simulink model "Drive_DC"  (R2022b)
settings: Solver=VariableStepAuto  StartTime=0.0  StopTime=13  MaxStep=1e-5  RelTol=1e-3
undefined symbols (not defined in the file or in its folder): DiscIntNeverNeededParam, sigbuilder_block
libraries: spsMeanLib x6, slpidlib x5, simulink_extras x5, spsSawtoothGeneratorLib x4, simulink x2, pid_lib x1, spspowerguiLib x1
(part 2 of 2)

== system Drive_DC/Dual_Rectifier_Control/Speed_Control ==
  note: PI_system3
  In1 : Inport
  In2 : Inport  Port=2
  AND : Logic  Operator=NAND  AllPortsSameDT=off  OutDataTypeStr=boolean
  Discrete-Time Integrator : DiscreteIntegrator  SampleTime=-1  ICPrevOutput=DiscIntNeverNeededParam  ICPrevScaledInput=DiscIntNeverNeededParam
  Equal : RelationalOperator  Operator=~=  OutDataTypeStr=boolean  RndMeth=Simplest  InputSameDT=off
  Equal1 : RelationalOperator  Operator===  OutDataTypeStr=boolean  RndMeth=Simplest  InputSameDT=off
  KI : Gain  Gain=0.5
  Kp : Gain  Gain=0.5
  PID Controller : slpidlib/PID Controller  Commented=on  Controller=PI  Form=Parallel  TimeDomain=Continuous-time  UseExternalTs=off  SampleTime=-1  IntegratorMethod=Forward Euler  FilterMethod=Forward Euler  ControllerParametersSource=internal  P=0.5  I=0.5  UseKiTs=off  D=0  N=100  UseFilter=on  TunerSelectOption=Transfer Function Based (PID Tuner App)  InitialConditionSource=internal  InitialConditionForIntegrator=0  InitialConditionForFilter=0  DifferentiatorICPrevScaledInput=0  ExternalReset=none  TrackingMode=off  Kt=1  LimitOutput=on  SatLimitsSource=internal  UpperSaturationLimit=(30*746)/(1740*pi/30)  LowerSaturationLimit=-(30*746)/(1740*pi/30)  LinearizeAsGain=on  AntiWindupMode=clamping  Kb=1  LimitIntegrator=off  UpperIntegratorSaturationLimit=inf  LowerIntegratorSaturationLimit=-inf  POutMin=[]  POutMax=[]  IOutMin=[]  IOutMax=[]  DOutMin=[]  DOutMax=[]  NOutMin=[]  NOutMax=[]  SumOutMin=[]  SumOutMax=[]  SaturationOutMin=[]  SaturationOutMax=[]  PParamMin=[]  PParamMax=[]  IParamMin=[]  IParamMax=[]  DParamMin=[]  DParamMax=[]  NParamMin=[]  NParamMax=[]  KbParamMin=[]  KbParamMax=[]  KtParamMin=[]  KtParamMax=[]  KbOutMin=[]  KbOutMax=[]  KtOutMin=[]  KtOutMax=[]  IntegratorOutMin=[]  IntegratorOutMax=[]  FilterOutMin=[]  FilterOutMax=[]  SumI1OutMin=[]  SumI1OutMax=[]  SumI2OutMin=[]  SumI2OutMax=[]  SumI3OutMin=[]  SumI3OutMax=[]  SumI4OutMin=[]  SumI4OutMax=[]  SumDOutMin=[]  SumDOutMax=[]  DifferentiatorOutMin=[]  DifferentiatorOutMax=[]  FilterDiffOutCoefMin=[]  FilterDiffOutCoefMax=[]  ReciprocalOutMin=[]  ReciprocalOutMax=[]  SumDenOutMin=[]  SumDenOutMax=[]  SumNumOutMin=[]  SumNumOutMax=[]  DivideOutMin=[]  DivideOutMax=[]  UdiffTsProdOutMin=[]  UdiffTsProdOutMax=[]  NTsProdOutMin=[]  NTsProdOutMax=[]  UintegralTsProdOutMin=[]  UintegralTsProdOutMax=[]  UngainTsProdOutMin=[]  UngainTsProdOutMax=[]  ClampingZeroOutDataTypeStr=Inherit: Inherit via back propagation  ClampingZeroOutMin=[]  ClampingZeroOutMax=[]  FilterDenConstantOutDataTypeStr=Inherit: Inherit via back propagation  FilterDenConstantOutMin=[]  FilterDenConstantOutMax=[]  PCopyOutDataTypeStr=Inherit: Inherit via back propagation  PCopyOutMin=[]  PCopyOutMax=[]  NCopyOutDataTypeStr=Inherit: Inherit via back propagation  NCopyOutMin=[]  NCopyOutMax=[]  IntegratorContinuousStateAttributes=''  IntegratorStateMustResolveToSignalObject=off  IntegratorRTWStateStorageClass=Auto  FilterContinuousStateAttributes=''  FilterStateMustResolveToSignalObject=off  FilterRTWStateStorageClass=Auto  ParallelPVariant=InternalParameters  IdealPVariant=Disabled  IVariant=InternalParameters  DVariant=Disabled  IntegratorVariant=Continuous  SatVariant=Enabled  AWVariant=ContClampingParallel  PCopyVariant=Disabled  TRVariant=Disabled  FdbkBlocksVariant=Forward  IdealPFdbkVariant=Disabled  SatFdbkVariant=Disabled  DerivativeFilterVariant=Disabled  NVariant=Disabled  NCopyVariant=Disabled_SignalSpec  FilterICVariant=Disabled  IntegratorICVariant=InternalICs  ExternalResetVariant=Disabled  TRSumVariant=Passthrough  SumFdbkVariant=Disabled  SumVariant=Sum_PI  TsampFilterVariant=InternalTs  TsampNgainVariant=Passthrough  TsampIntegralVariant=Passthrough  ExternalSaturationOutDataTypeStr=Inherit: Same as second input
  Product : Product
  Saturation1 : Saturate  UpperLimit=(30*746)/(1740*pi/30)  LowerLimit=-(30*746)/(1740*pi/30)
  Sign : Signum
  Sign1 : Signum
  Sum : Sum  Inputs=|+-
  Sum2 : Sum  Inputs=|++
  Unit Delay : UnitDelay  SampleTime=-1  HasFrameUpgradeWarning=on
  Unit Delay1 : UnitDelay  SampleTime=-1  HasFrameUpgradeWarning=on
  Tref : Outport
  wires:
  In2/1 -> Sum/2
  In1/1 -> Sum/1
  Discrete-Time Integrator/1 -> Sum2/1
  Kp/1 -> Sum2/2
  KI/1 -> Discrete-Time Integrator/1
  Sum2/1 -> Saturation1/1, Unit Delay/1
  Saturation1/1 -> Tref/1, Unit Delay1/1
  Sign/1 -> Equal1/2
  Sign1/1 -> Equal1/1
  Equal1/1 -> AND/1
  Equal/1 -> AND/2
  Unit Delay/1 -> Equal/1, Sign/1
  Product/1 -> KI/1
  Unit Delay1/1 -> Equal/2
  AND/1 -> Product/1
  Sum/1 -> Kp/1, Sign1/1, Product/2

== system Drive_DC/Dual_Rectifier_Control/Subsystem5 ==
  Va : Inport
  Vf : Inport  Port=2
  Tl : Inport  Port=3
  Gain : Gain  Gain=Ra
  Gain1 : Gain  Gain=k
  Gain2 : Gain  Gain=1/La
  Gain3 : Gain  Gain=Rf
  Gain4 : Gain  Gain=1/Lf
  Gain5 : Gain  Gain=k
  Gain6 : Gain  Gain=1/J
  Integrator : Integrator
  Integrator1 : Integrator
  Integrator2 : Integrator
  Subtract : Sum  Inputs=+--
  Subtract1 : Sum  Inputs=+-
  Subtract2 : Sum  Inputs=+-
  Ia : Outport
  If : Outport  Port=2
  Te : Outport  Port=3
  Wm : Outport  Port=4
  wires:
  Gain6/1 -> Integrator2/1
  Subtract2/1 -> Gain6/1
  Tl/1 -> Subtract2/2
  Gain5/1 -> Te/1, Subtract2/1
  Gain3/1 -> Subtract1/2
  Integrator1/1 -> If/1, Gain3/1
  Subtract1/1 -> Gain4/1
  Gain4/1 -> Integrator1/1
  Vf/1 -> Subtract1/1
  Gain2/1 -> Integrator/1
  Subtract/1 -> Gain2/1
  Gain1/1 -> Subtract/3
  Integrator2/1 -> Wm/1, Gain1/1
  Gain/1 -> Subtract/2
  Va/1 -> Subtract/1
  Integrator/1 -> Gain/1, Ia/1, Gain5/1

== system Drive_DC/Subsystem4/Subsystem ==
  Va : Inport
  W : Inport  Port=2
  Gain : Gain  Gain=Ra
  Gain1 : Gain  Gain=k
  Gain2 : Gain  Gain=1/La
  Integrator : Integrator
  Subtract : Sum  Inputs=+--
  Ia : Outport
  wires:
  Subtract/1 -> Gain2/1
  Integrator/1 -> Ia/1, Gain/1
  Va/1 -> Subtract/1
  Gain/1 -> Subtract/2
  Gain2/1 -> Integrator/1
  Gain1/1 -> Subtract/3
  W/1 -> Gain1/1

== system Drive_DC/Subsystem4/Subsystem1 ==
  Ia : Inport
  Gain5 : Gain  Gain=k
  Te : Outport
  wires:
  Gain5/1 -> Te/1
  Ia/1 -> Gain5/1

== system Drive_DC/Subsystem4/Subsystem3 ==
  In1 : Inport
  Gain3 : Gain  Gain=Rf
  Gain4 : Gain  Gain=1/Lf
  Integrator1 : Integrator
  Subtract1 : Sum  Inputs=+-
  Out1 : Outport
  wires:
  Subtract1/1 -> Gain4/1
  In1/1 -> Subtract1/1
  Integrator1/1 -> Out1/1, Gain3/1
  Gain3/1 -> Subtract1/2
  Gain4/1 -> Integrator1/1

== system Drive_DC/Chopper_Bipolar_Control/Rectifer_3/If Action Subsystem ==
  In1 : Inport
  Action Port : ActionPort  ActionPortLabel=if((u1 >= u2) & (u1 <= pi))
  Out1 : Outport
  wires:
  In1/1 -> Out1/1

== system Drive_DC/Chopper_Bipolar_Control/Rectifer_3/If Action Subsystem1 ==
  In1 : Inport
  Action Port : ActionPort  ActionPortLabel=elseif((u1 >= u3) & (u1 <= u4))
  Out1 : Outport
  wires:
  In1/1 -> Out1/1

== system Drive_DC/Chopper_Bipolar_Control/Rectifer_3/If Action Subsystem2 ==
  In1 : Inport
  Action Port : ActionPort  ActionPortLabel=else
  Out1 : Outport
  wires:
  In1/1 -> Out1/1

== system Drive_DC/Chopper_Unipolar_Control/Rectifer_3/If Action Subsystem ==
  In1 : Inport
  Action Port : ActionPort  ActionPortLabel=if((u1 >= u2) & (u1 <= pi))
  Out1 : Outport
  wires:
  In1/1 -> Out1/1

== system Drive_DC/Chopper_Unipolar_Control/Rectifer_3/If Action Subsystem1 ==
  In1 : Inport
  Action Port : ActionPort  ActionPortLabel=elseif((u1 >= u3) & (u1 <= u4))
  Out1 : Outport
  wires:
  In1/1 -> Out1/1

== system Drive_DC/Chopper_Unipolar_Control/Rectifer_3/If Action Subsystem2 ==
  In1 : Inport
  Action Port : ActionPort  ActionPortLabel=else
  Out1 : Outport
  wires:
  In1/1 -> Out1/1

== system Drive_DC/Dual_Rectifier_Control/Rectifer_3/If Action Subsystem ==
  In1 : Inport
  Action Port : ActionPort  ActionPortLabel=if((u1 >= u2) & (u1 <= pi))
  Out1 : Outport
  wires:
  In1/1 -> Out1/1

== system Drive_DC/Dual_Rectifier_Control/Rectifer_3/If Action Subsystem1 ==
  In1 : Inport
  Action Port : ActionPort  ActionPortLabel=elseif((u1 >= u3) & (u1 <= u4))
  Out1 : Outport
  wires:
  In1/1 -> Out1/1

== system Drive_DC/Dual_Rectifier_Control/Rectifer_3/If Action Subsystem2 ==
  In1 : Inport
  Action Port : ActionPort  ActionPortLabel=else
  Out1 : Outport
  wires:
  In1/1 -> Out1/1

== system Drive_DC/Dual_Rectifier_Control/Rectifer_4/If Action Subsystem ==
  In1 : Inport
  Action Port : ActionPort  ActionPortLabel=if((u1 >= u2) & (u1 <= pi))
  Out1 : Outport
  wires:
  In1/1 -> Out1/1

== system Drive_DC/Dual_Rectifier_Control/Rectifer_4/If Action Subsystem1 ==
  In1 : Inport
  Action Port : ActionPort  ActionPortLabel=elseif((u1 >= u3) & (u1 <= u4))
  Out1 : Outport
  wires:
  In1/1 -> Out1/1

== system Drive_DC/Dual_Rectifier_Control/Rectifer_4/If Action Subsystem2 ==
  In1 : Inport
  Action Port : ActionPort  ActionPortLabel=else
  Out1 : Outport
  wires:
  In1/1 -> Out1/1
